simulink library "Lib_Piccolo"  (R2018b)
settings: Solver=VariableStepAuto  StartTime=0.0  StopTime=10.0  RelTol=1e-3
values from neighbouring files (symbols this model uses):
  AccelErrInt2Brakes = 0.15    [SimulationControlConfig16P.m]    (also in SimulationControlConfig16P_LEGACY.m; SimulationControlConfigTAILLESS.m = 0.2; SimulationControlConfigUTAIL.m = 0.2)
  AileronMax = 25    [SimulationControlConfig16P.m]    (also in SimulationControlConfig16P_LEGACY.m; SimulationControlConfigTAILLESS.m; SimulationControlConfigUTAIL.m)
  AileronPower = 0.00268    [SimulationControlConfig16P.m]    (also in SimulationControlConfig16P_LEGACY.m; SimulationControlConfigTAILLESS.m; SimulationControlConfigUTAIL.m)
  AileronSurfaceMax = 45    [SimulationControlConfig16P.m]    (also in SimulationControlConfig16P_LEGACY.m)
  AileronTrim = 0    [SimulationControlConfig16P.m]    (also in SimulationControlConfig16P_LEGACY.m; SimulationControlConfigTAILLESS.m; SimulationControlConfigUTAIL.m)
  Alt = 1000 + TerrainHeight    [SimulationStateConfig.m]
  AltCruise_m = testPlans(testIndx).terrainElevation * 0.3048 + 200    [SimulationControlConfig16P.m]    (also in SimulationControlConfigTAILLESS.m = 1083; SimulationControlConfigUTAIL.m = testPlans(testIndx).terrainElevation * 0.3048 + 152)
  AltitudeRate2PitchCmdIntegratorInit = 0.1    [SimulationControlPre.m]
  AltMax = 10000    [SimulationControlConfig16P.m]    (also in SimulationControlConfig16P_LEGACY.m; SimulationControlConfigTAILLESS.m; SimulationControlConfigUTAIL.m)
  AltMaxAccel = 1.25    [SimulationControlConfig16P.m]    (also in SimulationControlConfig16P_LEGACY.m = 0.9; SimulationControlConfigTAILLESS.m = 1.7; SimulationControlConfigUTAIL.m = 2)
  AltMin = 0    [SimulationControlConfig16P.m]    (also in SimulationControlConfig16P_LEGACY.m; SimulationControlConfigTAILLESS.m; SimulationControlConfigUTAIL.m)
  AltRateCmd2Pitch = 0.50    (= 0.5)    [SimulationControlConfig16P.m]    (also in SimulationControlConfig16P_LEGACY.m = 0.6; SimulationControlConfigTAILLESS.m = 0.2; SimulationControlConfigUTAIL.m = 0.3)
  AltRateError2Pitch = 0.40    (= 0.4)    [SimulationControlConfig16P.m]    (also in SimulationControlConfig16P_LEGACY.m; SimulationControlConfigTAILLESS.m = 0.55; SimulationControlConfigUTAIL.m = 0.55)
  AltRateErrorInt2Pitch = 0.50    (= 0.5)    [SimulationControlConfig16P.m]    (also in SimulationControlConfig16P_LEGACY.m = 0.45; SimulationControlConfigTAILLESS.m; SimulationControlConfigUTAIL.m = 0.75)
  AltRateLpfCutOff = 3    [SimulationControlConfig16P.m]    (also in SimulationControlConfig16P_LEGACY.m; SimulationControlConfigTAILLESS.m = 2; SimulationControlConfigUTAIL.m = 2)
  AutoNosegear2Rudder = 26    [SimulationControlConfig16P.m]    (also in SimulationControlConfig16P_LEGACY.m; SimulationControlConfigTAILLESS.m = 25.2; SimulationControlConfigUTAIL.m = 14)
  b = 5.54    [SimulationControlConfig16P.m]    (also in SimulationControlConfig16P_LEGACY.m; SimulationControlConfigTAILLESS.m = 2.37; SimulationControlConfigUTAIL.m = 2.37)
  Bank2AileronIntegratorInit = 0    [SimulationControlPre.m]
  BankMax_User = BankMax_User/180*pi    (= 0.523598775598)    [SimulationControlConfig16P.m]    (also in SimulationControlConfig16P_LEGACY.m; SimulationControlConfigTAILLESS.m = 0.610865238198; SimulationControlConfigUTAIL.m = 0.628318530718)
  baseLegFlaps = 20    [SimulationControlConfig16P.m]    (also in SimulationControlConfig16P_LEGACY.m = 0; SimulationControlConfigTAILLESS.m = 15; SimulationControlConfigUTAIL.m = 10)
  C = GeneticOpt.C    [SimulationCostFunction.m]
  c = Sw/b    (= 0.841696750903)    [SimulationControlConfig16P.m]    (also in SimulationControlConfig16P_LEGACY.m; SimulationControlConfigTAILLESS.m = 0.354008438819; SimulationControlConfigUTAIL.m = 0.354008438819)
  cell2WheelFactorMG = 5.98    [SimulationSensorConfig16P_LEGACY.m]
  cell2WheelFactorNG = 1    [SimulationSensorConfig16P_LEGACY.m]
  cellSatMaxMG = 15000    [SimulationSensorConfig16P.m]    (also in SimulationSensorConfig16P_LEGACY.m; SimulationSensorConfigTAILLESS7P.m; SimulationSensorConfigUTAIL7P.m)
  cellSatMaxNG = 1000    [SimulationSensorConfig16P.m]    (also in SimulationSensorConfig16P_LEGACY.m; SimulationSensorConfigTAILLESS7P.m; SimulationSensorConfigUTAIL7P.m)
  cellSatMinMG = -15000    [SimulationSensorConfig16P.m]    (also in SimulationSensorConfig16P_LEGACY.m; SimulationSensorConfigTAILLESS7P.m; SimulationSensorConfigUTAIL7P.m)
  cellSatMinNG = -1000    [SimulationSensorConfig16P.m]    (also in SimulationSensorConfig16P_LEGACY.m; SimulationSensorConfigTAILLESS7P.m; SimulationSensorConfigUTAIL7P.m)
  CL_Limit = CL_Max    (= 0.54)    [SimulationControlConfig16P.m]    (also in SimulationControlConfig16P_LEGACY.m; SimulationControlConfigTAILLESS.m; SimulationControlConfigUTAIL.m = 0.53)
  CL_Max = 0.54    [SimulationControlConfig16P.m]    (also in SimulationControlConfig16P_LEGACY.m; SimulationControlConfigTAILLESS.m; SimulationControlConfigUTAIL.m = 0.53)
  CL_Max_Nom = 0.465    [SimulationControlConfig16P.m]    (also in SimulationControlConfig16P_LEGACY.m; SimulationControlConfigTAILLESS.m = 0.39; SimulationControlConfigUTAIL.m)
  CL_Min = 0    [SimulationControlConfig16P.m]    (also in SimulationControlConfig16P_LEGACY.m; SimulationControlConfigTAILLESS.m; SimulationControlConfigUTAIL.m)
  ClimbMaxFraction = 0.35    [SimulationControlConfig16P.m]    (also in SimulationControlConfig16P_LEGACY.m = 0.24; SimulationControlConfigTAILLESS.m = 0.19; SimulationControlConfigUTAIL.m = 0.21)
  ClimboutMaxBank = 7.0    (= 7)    [SimulationControlConfig16P.m]    (also in SimulationControlConfig16P_LEGACY.m; SimulationControlConfigTAILLESS.m = 5; SimulationControlConfigUTAIL.m)
  ClimboutTimer = 7.0    (= 7)    [SimulationControlConfig16P.m]    (also in SimulationControlConfig16P_LEGACY.m; SimulationControlConfigTAILLESS.m; SimulationControlConfigUTAIL.m)
  dCl_per_dFlap = 0.005581818    [SimulationControlConfig16P.m]    (also in SimulationControlConfig16P_LEGACY.m = 0; SimulationControlConfigTAILLESS.m = 0; SimulationControlConfigUTAIL.m = 0)
  DecelerationCmd = 3.1    [SimulationControlConfig16P.m]    (also in SimulationControlConfig16P_LEGACY.m; SimulationControlConfigTAILLESS.m = 0.1; SimulationControlConfigUTAIL.m = 0.1)
  DeRotateLogicEndTimer = abs((NoseDownLimit_Deg-1)/DeRotateRamp_Dps)    [SimulationControlConfig16P.m]    (also in SimulationControlConfig16P_LEGACY.m; SimulationControlConfigTAILLESS.m; SimulationControlConfigUTAIL.m)
  DeRotateLogicHoldNoseUpTimer = 0.1    [SimulationControlConfig16P.m]    (also in SimulationControlConfig16P_LEGACY.m; SimulationControlConfigTAILLESS.m; SimulationControlConfigUTAIL.m)
  DeRotateLogicTimerTimeout = 2    [SimulationControlConfig16P.m]    (also in SimulationControlConfig16P_LEGACY.m; SimulationControlConfigTAILLESS.m; SimulationControlConfigUTAIL.m)
  DeRotateLowerCmdSaturation = 0    [SimulationControlConfig16P.m]    (also in SimulationControlConfig16P_LEGACY.m; SimulationControlConfigTAILLESS.m; SimulationControlConfigUTAIL.m)
  DeRotateRamp_Dps = 3    [SimulationControlConfig16P.m]    (also in SimulationControlConfig16P_LEGACY.m; SimulationControlConfigTAILLESS.m = 8; SimulationControlConfigUTAIL.m = 8)
  DeRotateUpperCmdSaturation = 7    [SimulationControlConfig16P.m]    (also in SimulationControlConfig16P_LEGACY.m; SimulationControlConfigTAILLESS.m; SimulationControlConfigUTAIL.m)
  DescentMaxFraction = 0.22    [SimulationControlConfig16P.m]    (also in SimulationControlConfig16P_LEGACY.m = 0.2; SimulationControlConfigTAILLESS.m = 0.17; SimulationControlConfigUTAIL.m = 0.17)
  DesktopSimTerrainOffset_m = 0.406    [SimulationAircraftConfig.m]
  downwindFlaps = 0    [SimulationControlConfig16P.m]    (also in SimulationControlConfig16P_LEGACY.m; SimulationControlConfigTAILLESS.m; SimulationControlConfigUTAIL.m)
  DP_init = 0.5*1.225*V_init^2    [SimulationControlConfig16P.m]    (also in SimulationControlConfig16P_LEGACY.m; SimulationControlConfigTAILLESS.m; SimulationControlConfigUTAIL.m)
  dscNoiseMG = 1    [SimulationSensorConfig16P_LEGACY.m]
  dscNoiseNG = 0.25    [SimulationSensorConfig16P_LEGACY.m]
  DSCnumBits = 24    [SimulationSensorConfig16P.m]    (also in SimulationSensorConfig16P_LEGACY.m; SimulationSensorConfigTAILLESS7P.m; SimulationSensorConfigUTAIL7P.m)
  DSCRangeMaxMG = 15000    [SimulationSensorConfig16P.m]    (also in SimulationSensorConfig16P_LEGACY.m; SimulationSensorConfigTAILLESS7P.m; SimulationSensorConfigUTAIL7P.m)
  DSCRangeMaxNG = 1000    [SimulationSensorConfig16P.m]    (also in SimulationSensorConfig16P_LEGACY.m; SimulationSensorConfigTAILLESS7P.m; SimulationSensorConfigUTAIL7P.m)
  DSCRangeMinMG = -15000    [SimulationSensorConfig16P.m]    (also in SimulationSensorConfig16P_LEGACY.m; SimulationSensorConfigTAILLESS7P.m; SimulationSensorConfigUTAIL7P.m)
  DSCRangeMinNG = -1000    [SimulationSensorConfig16P.m]    (also in SimulationSensorConfig16P_LEGACY.m; SimulationSensorConfigTAILLESS7P.m; SimulationSensorConfigUTAIL7P.m)
  dt = DLLSim.dt    [SimulationTimeStep.m]    (also in SimulationTrim.m = 0.02)
  EarlyTouchdownThreshold = 3.0    (= 3)    [SimulationControlConfig16P.m]    (also in SimulationControlConfig16P_LEGACY.m; SimulationControlConfigTAILLESS.m = 2.2; SimulationControlConfigUTAIL.m = 2.5)
  ElevatorDeflectionRate = 15    [SimulationControlConfig16P.m]    (also in SimulationControlConfig16P_LEGACY.m = 12; SimulationControlConfigTAILLESS.m = 10; SimulationControlConfigUTAIL.m = 12)
  ElevatorMax = 25    [SimulationControlConfig16P.m]    (also in SimulationControlConfig16P_LEGACY.m; SimulationControlConfigTAILLESS.m; SimulationControlConfigUTAIL.m)
  ElevatorPower = -0.002209    [SimulationControlConfig16P.m]    (also in SimulationControlConfig16P_LEGACY.m; SimulationControlConfigTAILLESS.m = -0.002956; SimulationControlConfigUTAIL.m = -0.00205983)
  ElevatorTrim = -3.5    [SimulationControlConfig16P.m]    (also in SimulationControlConfig16P_LEGACY.m; SimulationControlConfigTAILLESS.m = -6; SimulationControlConfigUTAIL.m = -8)
  elevonBias = 0    [SimulationControlConfig16P.m]    (also in SimulationControlConfig16P_LEGACY.m; SimulationControlConfigTAILLESS.m; SimulationControlConfigUTAIL.m)
  Enable_TAS_Protection = 0    [SimulationControlConfig16P.m]    (also in SimulationControlConfig16P_LEGACY.m; SimulationControlConfigTAILLESS.m; SimulationControlConfigUTAIL.m)
  EnableCrossTrackAbort = 1    [SimulationControlConfig16P.m]    (also in SimulationControlConfigTAILLESS.m; SimulationControlConfigUTAIL.m)
  EnergyBandwidth = 0.02    [SimulationControlConfig16P.m]    (also in SimulationControlConfig16P_LEGACY.m; SimulationControlConfigTAILLESS.m = 0.06; SimulationControlConfigUTAIL.m = 0.06)
  EngineLhFuelCut = 0    [SimulationAircraftConfig.m]
  EngineRhFuelCut = 0    [SimulationAircraftConfig.m]
  FastThrottleRate = 0.075    [SimulationControlConfig16P.m]    (also in SimulationControlConfig16P_LEGACY.m = 0.05; SimulationControlConfigTAILLESS.m = 0.1; SimulationControlConfigUTAIL.m = 0.1)
  FilterWarmUpTime = 2    [SimulationSensorConfig16P.m]    (also in SimulationSensorConfig16P_LEGACY.m; SimulationSensorConfigTAILLESS7P.m; SimulationSensorConfigUTAIL7P.m)
  finalApproachFlaps = 20    [SimulationControlConfig16P.m]    (also in SimulationControlConfig16P_LEGACY.m = 0; SimulationControlConfigTAILLESS.m = 22; SimulationControlConfigUTAIL.m = 10)
  FinalDescentSlope_Deg = testPlans(testIndx).descentSlope    [SimulationControlConfig16P.m]    (also in SimulationControlConfig16P_LEGACY.m; SimulationControlConfigTAILLESS.m; SimulationControlConfigUTAIL.m)
  flapMax = 0    [SimulationControlConfig16P.m]    (also in SimulationControlConfig16P_LEGACY.m; SimulationControlConfigTAILLESS.m; SimulationControlConfigUTAIL.m)
  flapRate = 7.5    [SimulationControlConfig16P.m]    (also in SimulationControlConfig16P_LEGACY.m; SimulationControlConfigTAILLESS.m = 6.6; SimulationControlConfigUTAIL.m)
  FlareHeight = 5    [SimulationControlConfig16P.m]    (also in SimulationControlConfig16P_LEGACY.m = 4.8; SimulationControlConfigTAILLESS.m = 2.5; SimulationControlConfigUTAIL.m = 2)
  FlareVerticalRate_mps = -0.4    [SimulationControlConfig16P.m]    (also in SimulationControlConfig16P_LEGACY.m = -0.5; SimulationControlConfigTAILLESS.m = -0.15; SimulationControlConfigUTAIL.m = -0.15)
  Fp_Aileron = 0.55*2*pi*RollRateLpfCutoff*dt    [SimulationControlConfig16P.m]    (also in SimulationControlConfig16P_LEGACY.m; SimulationControlConfigTAILLESS.m; SimulationControlConfigUTAIL.m)
  Fp_Alt = 0.55*AltBandwidth    (= 0.099)    [SimulationControlConfig16P.m]    (also in SimulationControlConfig16P_LEGACY.m; SimulationControlConfigTAILLESS.m = 0.587477826221; SimulationControlConfigUTAIL.m = 0.69115038379)
  Fp_AltRate = 0.55*2*pi*AltRateLpfCutOff*dt    [SimulationControlConfig16P.m]    (also in SimulationControlConfig16P_LEGACY.m; SimulationControlConfigTAILLESS.m; SimulationControlConfigUTAIL.m)
  Fp_Elevator = 0.55*2*pi*PitchRateLpfCutoff*dt    [SimulationControlConfig16P.m]    (also in SimulationControlConfig16P_LEGACY.m; SimulationControlConfigTAILLESS.m; SimulationControlConfigUTAIL.m)
  Fp_Energy = 0.55*2*pi*EnergyBandwidth    (= 0.069115038379)    [SimulationControlConfig16P.m]    (also in SimulationControlConfig16P_LEGACY.m; SimulationControlConfigTAILLESS.m = 0.207345115137; SimulationControlConfigUTAIL.m = 0.207345115137)
  Fp_Energy2 = 0.55*2*pi*EnergyBandwidth*dt    [SimulationControlConfig16P.m]    (also in SimulationControlConfig16P_LEGACY.m; SimulationControlConfigTAILLESS.m; SimulationControlConfigUTAIL.m)
  Fp_Pitch = 0.55*2*pi*PitchBandwidth    (= 2.76460153516)    [SimulationControlConfig16P.m]    (also in SimulationControlConfig16P_LEGACY.m = 3.11017672705; SimulationControlConfigTAILLESS.m = 3.80132711084; SimulationControlConfigUTAIL.m = 2.41902634326)
  Fp_Pitch_2 = 0.55*2*pi*PitchBandwidth*dt    [SimulationControlConfig16P.m]    (also in SimulationControlConfig16P_LEGACY.m; SimulationControlConfigTAILLESS.m; SimulationControlConfigUTAIL.m)
  Fp_Roll = RollBandwidth^2    (= 1)    [SimulationControlConfig16P.m]    (also in SimulationControlConfig16P_LEGACY.m = 1.44; SimulationControlConfigTAILLESS.m; SimulationControlConfigUTAIL.m)
  Fp_Rudder = 0.55*2*pi*YawRateLpfCutoff*dt    [SimulationControlConfig16P.m]    (also in SimulationControlConfig16P_LEGACY.m; SimulationControlConfigTAILLESS.m; SimulationControlConfigUTAIL.m)
  Fp_TAS = 0.55*2*pi*TASBandwidth    (= 0.103672557568)    [SimulationControlConfig16P.m]    (also in SimulationControlConfig16P_LEGACY.m; SimulationControlConfigTAILLESS.m = 0.172787595947; SimulationControlConfigUTAIL.m = 0.172787595947)
  Fp_TAS_Filter = 2*pi*TasLpfCutoff*dt    [SimulationControlConfig16P.m]    (also in SimulationControlConfig16P_LEGACY.m; SimulationControlConfigTAILLESS.m; SimulationControlConfigUTAIL.m)
  Fp_Turn = 0.55*2*pi*TurnErrLPFcutoff    (= 0.0345575191895)    [SimulationControlConfig16P.m]    (also in SimulationControlConfig16P_LEGACY.m; SimulationControlConfigTAILLESS.m = 0.172787595947; SimulationControlConfigUTAIL.m = 0.172787595947)
  Fp_TurnDerr = 0.55*2*pi*TurnDerivativeLPFcutoff    (= 0.0345575191895)    [SimulationControlConfig16P.m]    (also in SimulationControlConfig16P_LEGACY.m; SimulationControlConfigTAILLESS.m = 0.172787595947; SimulationControlConfigUTAIL.m = 0.172787595947)
  FTV = 3    [SimulationAircraftConfig.m]
  ftvStaticPositionError = 1/1.18    (= 0.847457627119)    [SimulationSensorConfig16P.m]    (also in SimulationSensorConfig16P_LEGACY.m; SimulationSensorConfigTAILLESS7P.m = 1; SimulationSensorConfigUTAIL7P.m = 1)
  g = 9.81    [SimulationStateConfig.m]
  GustSpd_Kts = testPlans(testIndx).gustSpd    [SimulationStateConfig.m]
  GustTriggerVal = testPlans(testIndx).gustTriggerVal    [SimulationStateConfig.m]
  HeadingErr2TurnRate = 0.5    [SimulationControlConfig16P.m]    (also in SimulationControlConfig16P_LEGACY.m; SimulationControlConfigTAILLESS.m; SimulationControlConfigUTAIL.m)
  HeadingErrDer2TurnRate = 0.3    [SimulationControlConfig16P.m]    (also in SimulationControlConfig16P_LEGACY.m; SimulationControlConfigTAILLESS.m; SimulationControlConfigUTAIL.m)
  IASbounce = IASstall*0.8    [SimulationControlPre.m]
  IAScruiseCMD = sqrt(2*m*9.81/(1.225*Sw*CL_cruise))    [SimulationControlConfig16P.m]    (also in SimulationControlConfig16P_LEGACY.m; SimulationControlConfigTAILLESS.m; SimulationControlConfigUTAIL.m)
  IASfinalCMD = 1.12 * IASmin    [SimulationControlConfig16P.m]    (also in SimulationControlConfig16P_LEGACY.m = 1.10 * IASmin; SimulationControlConfigTAILLESS.m = 1.10 * IASmin; SimulationControlConfigUTAIL.m = 1.15 * IASmin)
  IASflareCMD = IASstall    [SimulationControlConfig16P.m]    (also in SimulationControlConfig16P_LEGACY.m; SimulationControlConfigTAILLESS.m; SimulationControlConfigUTAIL.m)
  IASmax = 64    [SimulationControlConfig16P.m]    (also in SimulationControlConfig16P_LEGACY.m = 46; SimulationControlConfigTAILLESS.m = 38.58; SimulationControlConfigUTAIL.m = 35)
  IASmin = sqrt(2*m*9.81/(1.225*Sw*0.9*CL_Max_Nom))    [SimulationControlConfig16P.m]    (also in SimulationControlConfig16P_LEGACY.m; SimulationControlConfigTAILLESS.m; SimulationControlConfigUTAIL.m)
  IASshortCMD = IASstall    [SimulationControlConfig16P.m]    (also in SimulationControlConfig16P_LEGACY.m; SimulationControlConfigTAILLESS.m; SimulationControlConfigUTAIL.m)
  IASstall = sqrt(2*m*9.81/(1.225*Sw*CL_Max))    [SimulationControlConfig16P.m]    (also in SimulationControlConfig16P_LEGACY.m; SimulationControlConfigTAILLESS.m; SimulationControlConfigUTAIL.m)
  inFlight = 1    [SimulationControlConfig16P.m]    (also in SimulationControlConfigTAILLESS.m; SimulationControlConfigUTAIL.m)
  JetCatOffset = 5    [SimulationControlConfig16P.m]    (also in SimulationControlConfig16P_LEGACY.m)
  LaunchRollingElevator = -1.5    [SimulationControlConfig16P.m]    (also in SimulationControlConfig16P_LEGACY.m; SimulationControlConfigTAILLESS.m = 1; SimulationControlConfigUTAIL.m = 1)
  ldg_NosegearMax = 10    [SimulationControlConfig16P.m]    (also in SimulationControlConfig16P_LEGACY.m; SimulationControlConfigTAILLESS.m; SimulationControlConfigUTAIL.m)
  ldg_TrackVyErrInt2Nosegear = 0.1250    (= 0.125)    [SimulationControlConfig16P.m]    (also in SimulationControlConfig16P_LEGACY.m; SimulationControlConfigTAILLESS.m = 0.00714285714286; SimulationControlConfigUTAIL.m = 0.00714285714286)
  ldg_TrackVyErrPro2Nosegear = 0.35    [SimulationControlConfig16P.m]    (also in SimulationControlConfig16P_LEGACY.m; SimulationControlConfigTAILLESS.m = 0.0546666666667; SimulationControlConfigUTAIL.m = 0.0546666666667)
  ldg_TrackY2Vy = 0.07    [SimulationControlConfig16P.m]    (also in SimulationControlConfig16P_LEGACY.m; SimulationControlConfigTAILLESS.m = 0.17; SimulationControlConfigUTAIL.m = 0.17)
  ldg_Vy2NosegearScalingPower = 1.075    [SimulationControlConfig16P.m]    (also in SimulationControlConfig16P_LEGACY.m; SimulationControlConfigTAILLESS.m = 0.6; SimulationControlConfigUTAIL.m = 0.5)
  ldg_Y2VyScalingPower = 0.175    [SimulationControlConfig16P.m]    (also in SimulationControlConfig16P_LEGACY.m; SimulationControlConfigTAILLESS.m = 0; SimulationControlConfigUTAIL.m = 0)
  ldg_YawRate2Nosegear = 0.175    [SimulationControlConfig16P.m]    (also in SimulationControlConfig16P_LEGACY.m; SimulationControlConfigTAILLESS.m = 0.065; SimulationControlConfigUTAIL.m = 0.065)
  LiftSlope = 0.064285    [SimulationControlConfig16P.m]    (also in SimulationControlConfig16P_LEGACY.m; SimulationControlConfigTAILLESS.m = 0.058631; SimulationControlConfigUTAIL.m)
  LPFaileronInit = 0    [SimulationControlPre.m]
  LPFclestInit = 0    [SimulationControlPre.m]
  LPFenergyFFInit = 0    [SimulationControlPre.m]
  LPFtasInit = V_init + 2    [SimulationControlPre.m]
  LPFthrottleInit = ThrottleTrim    [SimulationControlPre.m]
  LPFturnErrInit = 0    [SimulationControlPre.m]
  ... (+115 more)
undefined symbols (not defined in the file or in its folder): abortFlag, alphaHPF, apmDelay, BRWNOUT, CRAWOR, CRAWUR, DiscIntNeverNeededParam, DLLSim, DLLSimStep, ECOMOR, ECOMUR, Fp_Tas, GustTrigger_HeightAgl_m, IPSTAT, LCINTEG, Ldg_Persist_Time, LOWER_FLAGS, MSG_ENABLE, NoiseStd, OLDVAL, OVERRIDE_ENABLE, OVERRIDE_VALUE, REBOOT, reversionEnable, revIASMax, revIASMin, revPitchMax, revPitchMin, revPitchRateMax, revRollMax, revRollRateMax, SAMPLE, SCALON, SensorModel, sigbuilder_block, Sim_Vx, Sim_Vy, Sim_Vz, Sim_Xpos, Sim_Ypos, Sim_Zpos, SYSOR, SYSUR, TARE, TEMPOR, TEMPUR, testIndx, testPlan, testPlans, Trim_piccoloInCmd, Trim_REFSI_FD_IN_nmodeCgShifterCmd_Ft, Trim_REFSI_FD_IN_nmodeFlapLhIBCmd_Deg, Trim_REFSI_FD_IN_nmodeFlapLhOBCmd_Deg, Trim_REFSI_FD_IN_nmodeFlapRhIBCmd_Deg, Trim_REFSI_FD_IN_nmodeFlapRhOBCmd_Deg, Trim_REFSI_FD_IN_nmodeSlatLhCmd_Deg, Trim_REFSI_FD_IN_nmodeSlatRhCmd_Deg, Trim_REFSI_FD_IN_nmodeSplrLhInbdCmd_Deg, Trim_REFSI_FD_IN_nmodeSplrLhOutbdCmd_Deg ... (+5)
libraries: simulink x866, aerolibconvert2 x60, $bdroot x52, aerolibatmos2 x5, dspswit3 x5, simulink_extras x4, dsparch4 x2, Lib_Piccolo_Alt x2, eeGeneralControl x1, dspindex x1
(part 42 of 44)

== system Lib_Piccolo/Ground Detection Systems/WoW Wrapper/Variant Subsystem/Load Cell WoW Model 20/WOW Module/Subsystem/Comms Timeout Logic ==
  MGR_STALE_LOAD : Inport  OutDataTypeStr=boolean
  MGL_STALE_LOAD : Inport  Port=2  OutDataTypeStr=boolean
  NG_STALE_LOAD : Inport  Port=3  OutDataTypeStr=boolean
  MGR_STALE_FLAG : Inport  Port=4  OutDataTypeStr=boolean
  MGL_STALE_FLAG : Inport  Port=5  OutDataTypeStr=boolean
  NG_STALE_FLAG : Inport  Port=6  OutDataTypeStr=boolean
  INIT : Inport  Port=7  OutDataTypeStr=boolean
  AND{,1..14} (15 alike) : Logic  IconShape=distinctive  AllPortsSameDT=off  OutDataTypeStr=boolean
  FLAG Timeout Counter : Subsystem
  FLAG Timeout Counter1 : $bdroot/Ground Detection Systems/WoW Wrapper/Variant Subsystem/Load Cell WoW Model 20/WOW Module/Subsystem/Comms Timeout Logic/FLAG Timeout Counter  SystemSampleTime=-1
  FLAG Timeout Counter2 : $bdroot/Ground Detection Systems/WoW Wrapper/Variant Subsystem/Load Cell WoW Model 20/WOW Module/Subsystem/Comms Timeout Logic/FLAG Timeout Counter  SystemSampleTime=-1
  LOAD Timeout Counter : Subsystem
  LOAD Timeout Counter1 : $bdroot/Ground Detection Systems/WoW Wrapper/Variant Subsystem/Load Cell WoW Model 20/WOW Module/Subsystem/Comms Timeout Logic/LOAD Timeout Counter  SystemSampleTime=-1
  LOAD Timeout Counter2 : $bdroot/Ground Detection Systems/WoW Wrapper/Variant Subsystem/Load Cell WoW Model 20/WOW Module/Subsystem/Comms Timeout Logic/LOAD Timeout Counter  SystemSampleTime=-1
  Latch : Subsystem
  Latch{1..5} (5 alike) : $bdroot/Ground Detection Systems/WoW Wrapper/Variant Subsystem/Load Cell WoW Model 20/WOW Module/Subsystem/Comms Timeout Logic/Latch  SystemSampleTime=-1
  NOT{,1..6} (7 alike) : Logic  Operator=NOT  IconShape=distinctive  AllPortsSameDT=off  OutDataTypeStr=boolean
  Reset Value Selector : Subsystem
  MGR_LOAD_TIMEOUT : Outport  OutDataTypeStr=boolean
  MGL_LOAD_TIMEOUT : Outport  Port=2  OutDataTypeStr=boolean
  NG_LOAD_TIMEOUT : Outport  Port=3  OutDataTypeStr=boolean
  MGR_FLAG_TIMEOUT : Outport  Port=4  OutDataTypeStr=boolean
  MGL_FLAG_TIMEOUT : Outport  Port=5  OutDataTypeStr=boolean
  NG_FLAG_TIMEOUT : Outport  Port=6  OutDataTypeStr=boolean
  MGR_ACTIVE : Outport  Port=7  OutDataTypeStr=boolean
  MGL_ACTIVE : Outport  Port=8  OutDataTypeStr=boolean
  NG_ACTIVE : Outport  Port=9  OutDataTypeStr=boolean
  wires:
  AND5/1 -> LOAD Timeout Counter1/1
  AND6/1 -> LOAD Timeout Counter2/1
  MGR_STALE_LOAD/1 -> NOT/1, AND4/1
  AND8/1 -> FLAG Timeout Counter1/1
  Reset Value Selector/1(Reset Value LOAD) -> LOAD Timeout Counter2/2, LOAD Timeout Counter1/2, LOAD Timeout Counter/2(x0)
  LOAD Timeout Counter2/1 -> NG_LOAD_TIMEOUT/1  "NG_LOAD_TIMEOUT"
  AND7/1 -> FLAG Timeout Counter/1(Trigger/!Rst)
  AND9/1 -> FLAG Timeout Counter2/1
  INIT/1 -> NOT1/1, Reset Value Selector/1(Init)
  AND4/1 -> LOAD Timeout Counter/1(Trigger/!Rst)
  Reset Value Selector/2(Reset Value FLAG) -> FLAG Timeout Counter2/2, FLAG Timeout Counter1/2, FLAG Timeout Counter/2(x0)
  FLAG Timeout Counter1/1 -> MGL_FLAG_TIMEOUT/1  "MGL_FLAG_TIMEOUT"
  FLAG Timeout Counter/1(TIMEOUT) -> MGR_FLAG_TIMEOUT/1  "MGR_FLAG_TIMEOUT"
  LOAD Timeout Counter1/1 -> MGL_LOAD_TIMEOUT/1  "MGL_LOAD_TIMEOUT"
  FLAG Timeout Counter2/1 -> NG_FLAG_TIMEOUT/1  "NG_FLAG_TIMEOUT"
  LOAD Timeout Counter/1(TIMEOUT) -> MGR_LOAD_TIMEOUT/1  "MGR_LOAD_TIMEOUT"
  NOT/1 -> AND1/1
  NOT2/1 -> AND2/1
  MGL_STALE_LOAD/1 -> NOT2/1, AND5/1
  NOT3/1 -> AND3/1
  NG_STALE_LOAD/1 -> NOT3/1, AND6/1
  NOT4/1 -> AND10/1
  MGR_STALE_FLAG/1 -> NOT4/1, AND7/1
  NOT5/1 -> AND11/1
  MGL_STALE_FLAG/1 -> NOT5/1, AND8/1
  NOT6/1 -> AND12/1
  NG_STALE_FLAG/1 -> NOT6/1, AND9/1
  NOT1/1 -> AND1/2, Latch/2(Enable/!Rst), AND4/2, AND2/2, Latch1/2, AND5/2, AND3/2, Latch2/2, AND6/2, AND10/2, Latch3/2, AND7/2, AND11/2, Latch4/2, AND8/2, AND12/2, Latch5/2, AND9/2
  AND1/1 -> Latch/1(D)
  AND2/1 -> Latch1/1
  AND3/1 -> Latch2/1
  AND10/1 -> Latch3/1
  Latch/1(Q_Latched) -> AND/1  "MGR_LOAD_ACTIVE"
  AND11/1 -> Latch4/1
  AND12/1 -> Latch5/1
  Latch1/1 -> AND13/1  "MGL_LOAD_ACTIVE"
  Latch2/1 -> AND14/1  "NG_LOAD_ACTIVE"
  Latch3/1 -> AND/2  "MGR_FLAG_ACTIVE"
  Latch4/1 -> AND13/2  "MGL_FLAG_ACTIVE"
  Latch5/1 -> AND14/2  "NG_FLAG_ACTIVE"
  AND/1 -> MGR_ACTIVE/1
  AND13/1 -> MGL_ACTIVE/1
  AND14/1 -> NG_ACTIVE/1

== system Lib_Piccolo/Ground Detection Systems/WoW Wrapper/Variant Subsystem/Load Cell WoW Model 20/WOW Module/Subsystem/Health Check ==
  PIC_AP_MODE : Inport  OutDataTypeStr=uint8
  MGR FLAG Word : Inport  Port=2  OutDataTypeStr=uint16
  MGR STAT Word : Inport  Port=3  OutDataTypeStr=uint16
  MGL FLAG Word : Inport  Port=4  OutDataTypeStr=uint16
  MGL STAT Word : Inport  Port=5  OutDataTypeStr=uint16
  NG FLAG Word : Inport  Port=6  OutDataTypeStr=uint16
  NG STAT Word : Inport  Port=7  OutDataTypeStr=uint16
  MGR_LOAD_TIMEOUT : Inport  Port=8  OutDataTypeStr=boolean
  MGL_LOAD_TIMEOUT : Inport  Port=9  OutDataTypeStr=boolean
  NG_LOAD_TIMEOUT : Inport  Port=10  OutDataTypeStr=boolean
  MGR_FLAG_TIMEOUT : Inport  Port=11  OutDataTypeStr=boolean
  MGL_FLAG_TIMEOUT : Inport  Port=12  OutDataTypeStr=boolean
  NG_FLAG_TIMEOUT : Inport  Port=13  OutDataTypeStr=boolean
  WOW_N : Inport  Port=14
  Bus Selector : BusSelector  OutputSignals=WOW_MGR_N,WOW_MGL_N,WOW_NG_N
  DSC FLAG Decode : Subsystem
  DSC STAT Decode : Subsystem
  MGL DSC Fail Logic : $bdroot/Ground Detection Systems/WoW Wrapper/Variant Subsystem/Load Cell WoW Model 20/WOW Module/Subsystem/Health Check/MGR DSC Fail Logic  SystemSampleTime=-1
  MGR DSC Fail Logic : Subsystem
  NG DSC Fail Logic : Subsystem
  MGR_FAIL : Outport  OutDataTypeStr=boolean
  MGL_FAIL : Outport  Port=2  OutDataTypeStr=boolean
  NG_FAIL : Outport  Port=3  OutDataTypeStr=boolean
  MGR_FLAGS : Outport  Port=4  OutDataTypeStr=Bus: FLAG_SIGNAL_BUS
  MGL_FLAGS : Outport  Port=5  OutDataTypeStr=Bus: FLAG_SIGNAL_BUS
  NG_FLAGS : Outport  Port=6  OutDataTypeStr=Bus: FLAG_SIGNAL_BUS
  MGR_HEALTH : Outport  Port=7  OutDataTypeStr=Bus: HEALTH_SIGNAL_BUS
  MGL_HEALTH : Outport  Port=8  OutDataTypeStr=Bus: HEALTH_SIGNAL_BUS
  NG_HEALTH : Outport  Port=9  OutDataTypeStr=Bus: HEALTH_SIGNAL_BUS
  MGR_STAT : Outport  Port=10  OutDataTypeStr=Bus: STAT_SIGNAL_BUS
  MGL_STAT : Outport  Port=11  OutDataTypeStr=Bus: STAT_SIGNAL_BUS
  NG_STAT : Outport  Port=12  OutDataTypeStr=Bus: STAT_SIGNAL_BUS
  wires:
  DSC FLAG Decode/1(MGR_FLAG_RESET) -> MGR DSC Fail Logic/4(FLAG_RESET)  "MGR_FLAG_RESET"
  NG FLAG Word/1 -> DSC FLAG Decode/3(NG FLAG Word)
  DSC FLAG Decode/6(NG_FLAGS) -> NG_FLAGS/1  "NG_FLAGS"
  DSC FLAG Decode/4(MGR_FLAGS) -> MGR_FLAGS/1  "MGR_FLAGS"
  DSC FLAG Decode/5(MGL_FLAGS) -> MGL_FLAGS/1  "MGL_FLAGS"
  MGL FLAG Word/1 -> DSC FLAG Decode/2(MGL FLAG Word)
  DSC FLAG Decode/2(MGL_FLAG_RESET) -> MGL DSC Fail Logic/4  "MGL_FLAG_RESET"
  DSC FLAG Decode/3(NG_FLAG_RESET) -> NG DSC Fail Logic/4(FLAG_RESET)  "NG_FLAG_RESET"
  MGR FLAG Word/1 -> DSC FLAG Decode/1(MGR FLAG Word)
  MGR_LOAD_TIMEOUT/1 -> MGR DSC Fail Logic/3(LOAD_TIMEOUT)
  MGL_LOAD_TIMEOUT/1 -> MGL DSC Fail Logic/3
  NG_LOAD_TIMEOUT/1 -> NG DSC Fail Logic/3(LOAD_TIMEOUT)
  MGR DSC Fail Logic/1(DSC_FAIL) -> MGR_FAIL/1  "MGR_DSC_FAIL"
  MGL DSC Fail Logic/1 -> MGL_FAIL/1  "MGL_DSC_FAIL"
  NG DSC Fail Logic/1(DSC_FAIL) -> NG_FAIL/1  "NG_DSC_FAIL"
  MGR DSC Fail Logic/2(MGR_HEALTH) -> MGR_HEALTH/1  "MGR_HEALTH"
  MGL DSC Fail Logic/2 -> MGL_HEALTH/1  "MGL_HEALTH"
  NG DSC Fail Logic/2(MGR_HEALTH) -> NG_HEALTH/1  "NG_HEALTH"
  WOW_N/1 -> Bus Selector/1
  Bus Selector/1 -> MGR DSC Fail Logic/2(WOW_N)  "<WOW_MGR_N>"
  Bus Selector/2 -> MGL DSC Fail Logic/2  "<WOW_MGL_N>"
  Bus Selector/3 -> NG DSC Fail Logic/2(WOW_N)  "<WOW_NG_N>"
  MGL STAT Word/1 -> DSC STAT Decode/2(MGL STAT Word)
  NG STAT Word/1 -> DSC STAT Decode/3(NG STAT Word)
  MGR STAT Word/1 -> DSC STAT Decode/1(MGR STAT Word)
  DSC STAT Decode/1(MGR_STAT) -> MGR_STAT/1
  DSC STAT Decode/2(MGL_STAT) -> MGL_STAT/1
  DSC STAT Decode/3(NG_STAT) -> NG_STAT/1
  PIC_AP_MODE/1 -> NG DSC Fail Logic/1(PIC_AP_MODE), MGL DSC Fail Logic/1, MGR DSC Fail Logic/1(PIC_AP_MODE)
  MGR_FLAG_TIMEOUT/1 -> MGR DSC Fail Logic/5(FLAG_TIMEOUT)
  MGL_FLAG_TIMEOUT/1 -> MGL DSC Fail Logic/5
  NG_FLAG_TIMEOUT/1 -> NG DSC Fail Logic/5(FLAG_TIMEOUT)

== system Lib_Piccolo/Ground Detection Systems/WoW Wrapper/Variant Subsystem/Load Cell WoW Model 20/WOW Module/T//O Configuration/Latch ==
  D : Inport
  Enable/!Rst : Inport  Port=2
  AND : Logic  IconShape=distinctive  AllPortsSameDT=off  OutDataTypeStr=boolean
  Constant : Constant  OutDataTypeStr=boolean
  OR : Logic  Operator=OR  IconShape=distinctive  AllPortsSameDT=off  OutDataTypeStr=boolean
  Switch : Switch  Criteria=u2 > Threshold  Threshold=0.5
  Unit Delay : UnitDelay  SampleTime=-1
  Q_Latched : Outport
  wires:
  Unit Delay/1 -> OR/2
  Switch/1 -> Q_Latched/1, Unit Delay/1
  D/1 -> Switch/3, OR/1
  OR/1 -> AND/1
  AND/1 -> Switch/2
  Enable/!Rst/1 -> AND/2
  Constant/1 -> Switch/1

== system Lib_Piccolo/Ground Detection Systems/WoW Wrapper/Variant Subsystem/Load Cell WoW Model 20/WOW Module/T//O Configuration/Latch Timer ==
  Enable/!Rst : Inport
  Compare To Constant1 : simulink/Logic and Bit Operations/Compare To Constant  relop=>  const=0  OutDataTypeStr=uint8
  Compare To Constant2 : simulink/Logic and Bit Operations/Compare To Constant  relop=>=  const=period  OutDataTypeStr=boolean
  Compare To Constant3 : simulink/Logic and Bit Operations/Compare To Constant  relop===  const=0  OutDataTypeStr=boolean
  Discrete-Time Integrator : DiscreteIntegrator  ExternalReset=level  SampleTime=-1  OutDataTypeStr=double  ICPrevOutput=DiscIntNeverNeededParam  ICPrevScaledInput=DiscIntNeverNeededParam
  Expired : Outport
  wires:
  Compare To Constant3/1 -> Discrete-Time Integrator/2
  Enable/!Rst/1 -> Compare To Constant3/1, Compare To Constant1/1
  Discrete-Time Integrator/1 -> Compare To Constant2/1
  Compare To Constant2/1 -> Expired/1
  Compare To Constant1/1 -> Discrete-Time Integrator/1

== system Lib_Piccolo/Ground Detection Systems/WoW Wrapper/Variant Subsystem/Load Cell WoW Model 20/WOW Module/T//O Configuration/Persistance Timer ==
  Enable/!Rst : Inport
  Compare To Constant1 : simulink/Logic and Bit Operations/Compare To Constant  relop=>  const=0  OutDataTypeStr=uint8
  Compare To Constant2 : simulink/Logic and Bit Operations/Compare To Constant  relop=>=  const=period  OutDataTypeStr=boolean
  Compare To Constant3 : simulink/Logic and Bit Operations/Compare To Constant  relop===  const=0  OutDataTypeStr=boolean
  Discrete-Time Integrator : DiscreteIntegrator  ExternalReset=level  SampleTime=-1  OutDataTypeStr=double  ICPrevOutput=DiscIntNeverNeededParam  ICPrevScaledInput=DiscIntNeverNeededParam
  Expired : Outport
  wires:
  Compare To Constant3/1 -> Discrete-Time Integrator/2
  Enable/!Rst/1 -> Compare To Constant3/1, Compare To Constant1/1
  Discrete-Time Integrator/1 -> Compare To Constant2/1
  Compare To Constant2/1 -> Expired/1
  Compare To Constant1/1 -> Discrete-Time Integrator/1

== system Lib_Piccolo/Ground Detection Systems/WoW Wrapper/Variant Subsystem/Load Cell WoW Model 1/Landing Configuration/Latch Timer Selection/Latch Timer Selection/Timer Select Latch ==
  D : Inport
  Enable/!Rst : Inport  Port=2
  AND : Logic  IconShape=distinctive  AllPortsSameDT=off  OutDataTypeStr=boolean
  Constant : Constant
  OR : Logic  Operator=OR  IconShape=distinctive  AllPortsSameDT=off  OutDataTypeStr=boolean
  Switch : Switch  Criteria=u2 > Threshold  Threshold=0.5
  Unit Delay : UnitDelay  SampleTime=-1
  Q_Latched : Outport
  wires:
  Unit Delay/1 -> OR/2
  Switch/1 -> Q_Latched/1, Unit Delay/1
  D/1 -> Switch/3, OR/1
  OR/1 -> AND/1
  AND/1 -> Switch/2
  Enable/!Rst/1 -> AND/2
  Constant/1 -> Switch/1

== system Lib_Piccolo/Ground Detection Systems/WoW Wrapper/Variant Subsystem/Load Cell WoW Model 1 16P5 AsFlown 2022/Landing Configuration/Latch Timer Selection/Latch Timer Selection/Timer Select Latch ==
  D : Inport
  Enable/!Rst : Inport  Port=2
  AND : Logic  IconShape=distinctive  AllPortsSameDT=off  OutDataTypeStr=boolean
  Constant : Constant
  OR : Logic  Operator=OR  IconShape=distinctive  AllPortsSameDT=off  OutDataTypeStr=boolean
  Switch : Switch  Criteria=u2 > Threshold  Threshold=0.5
  Unit Delay : UnitDelay  SampleTime=-1
  Q_Latched : Outport
  wires:
  Constant/1 -> Switch/1
  Enable/!Rst/1 -> AND/2
  AND/1 -> Switch/2
  OR/1 -> AND/1
  D/1 -> OR/1, Switch/3
  Switch/1 -> Unit Delay/1, Q_Latched/1
  Unit Delay/1 -> OR/2

== system Lib_Piccolo/Ground Detection Systems/WoW Wrapper/Variant Subsystem/Load Cell WoW Model 1 7P AsFlown/Landing Configuration/Latch Timer Selection/Latch Timer Selection/Timer Select Latch ==
  D : Inport
  Enable/!Rst : Inport  Port=2
  AND : Logic  IconShape=distinctive  AllPortsSameDT=off  OutDataTypeStr=boolean
  Constant : Constant
  OR : Logic  Operator=OR  IconShape=distinctive  AllPortsSameDT=off  OutDataTypeStr=boolean
  Switch : Switch  Criteria=u2 > Threshold  Threshold=0.5
  Unit Delay : UnitDelay  SampleTime=-1
  Q_Latched : Outport
  wires:
  Unit Delay/1 -> OR/2
  Switch/1 -> Q_Latched/1, Unit Delay/1
  D/1 -> Switch/3, OR/1
  OR/1 -> AND/1
  AND/1 -> Switch/2
  Enable/!Rst/1 -> AND/2
  Constant/1 -> Switch/1

== system Lib_Piccolo/Ground Detection Systems/WoW Wrapper/Variant Subsystem/Load Cell WoW Model 18/Subsystem/Landing Configuration/Latching Logic/Latch ==
  D : Inport
  Enable/!Rst : Inport  Port=2
  AND : Logic  IconShape=distinctive  AllPortsSameDT=off  OutDataTypeStr=boolean
  Constant : Constant  OutDataTypeStr=boolean
  OR : Logic  Operator=OR  IconShape=distinctive  AllPortsSameDT=off  OutDataTypeStr=boolean
  Switch : Switch  Criteria=u2 > Threshold  Threshold=0.5
  Unit Delay : UnitDelay  SampleTime=-1
  Q_Latched : Outport
  wires:
  Constant/1 -> Switch/1
  Enable/!Rst/1 -> AND/2
  AND/1 -> Switch/2
  OR/1 -> AND/1
  D/1 -> OR/1, Switch/3
  Switch/1 -> Unit Delay/1, Q_Latched/1
  Unit Delay/1 -> OR/2

== system Lib_Piccolo/Ground Detection Systems/WoW Wrapper/Variant Subsystem/Load Cell WoW Model 18/Subsystem/Landing Configuration/Latching Logic/Primary Latch Timer ==
  Enable/!Rst : Inport
  Compare To Constant1 : simulink/Logic and Bit Operations/Compare To Constant  relop=>  const=0  OutDataTypeStr=uint8
  Compare To Constant2 : simulink/Logic and Bit Operations/Compare To Constant  relop=>=  const=period  OutDataTypeStr=boolean
  Compare To Constant3 : simulink/Logic and Bit Operations/Compare To Constant  relop===  const=0  OutDataTypeStr=boolean
  Discrete-Time Integrator : DiscreteIntegrator  ExternalReset=level  SampleTime=-1  OutDataTypeStr=double  ICPrevOutput=DiscIntNeverNeededParam  ICPrevScaledInput=DiscIntNeverNeededParam
  Expired : Outport
  wires:
  Compare To Constant1/1 -> Discrete-Time Integrator/1
  Compare To Constant2/1 -> Expired/1
  Discrete-Time Integrator/1 -> Compare To Constant2/1
  Enable/!Rst/1 -> Compare To Constant1/1, Compare To Constant3/1
  Compare To Constant3/1 -> Discrete-Time Integrator/2

== system Lib_Piccolo/Ground Detection Systems/WoW Wrapper/Variant Subsystem/Load Cell WoW Model 18/Subsystem/Landing Configuration/Timeout Logic/1-Wheel Timeout ==
  Enable/!Rst : Inport
  Compare To Constant1 : simulink/Logic and Bit Operations/Compare To Constant  relop=>  const=0  OutDataTypeStr=uint8
  Compare To Constant2 : simulink/Logic and Bit Operations/Compare To Constant  relop=>=  const=period  OutDataTypeStr=boolean
  Compare To Constant3 : simulink/Logic and Bit Operations/Compare To Constant  relop===  const=0  OutDataTypeStr=boolean
  Discrete-Time Integrator : DiscreteIntegrator  ExternalReset=level  SampleTime=-1  OutDataTypeStr=double  ICPrevOutput=DiscIntNeverNeededParam  ICPrevScaledInput=DiscIntNeverNeededParam
  Expired : Outport
  wires:
  Compare To Constant1/1 -> Discrete-Time Integrator/1
  Compare To Constant2/1 -> Expired/1
  Discrete-Time Integrator/1 -> Compare To Constant2/1
  Enable/!Rst/1 -> Compare To Constant1/1, Compare To Constant3/1
  Compare To Constant3/1 -> Discrete-Time Integrator/2

== system Lib_Piccolo/Ground Detection Systems/WoW Wrapper/Variant Subsystem/Load Cell WoW Model 20/WOW Module/Landing Configuration/Latching Logic/Latch ==
  D : Inport
  Enable/!Rst : Inport  Port=2
  AND : Logic  IconShape=distinctive  AllPortsSameDT=off  OutDataTypeStr=boolean
  Constant : Constant  OutDataTypeStr=boolean
  OR : Logic  Operator=OR  IconShape=distinctive  AllPortsSameDT=off  OutDataTypeStr=boolean
  Switch : Switch  Criteria=u2 > Threshold  Threshold=0.5
  Unit Delay : UnitDelay  SampleTime=-1
  Q_Latched : Outport
  wires:
  Constant/1 -> Switch/1
  Enable/!Rst/1 -> AND/2
  AND/1 -> Switch/2
  OR/1 -> AND/1
  D/1 -> OR/1, Switch/3
  Switch/1 -> Unit Delay/1, Q_Latched/1
  Unit Delay/1 -> OR/2

== system Lib_Piccolo/Ground Detection Systems/WoW Wrapper/Variant Subsystem/Load Cell WoW Model 20/WOW Module/Landing Configuration/Latching Logic/Primary Latch Timer ==
  Enable/!Rst : Inport
  Compare To Constant1 : simulink/Logic and Bit Operations/Compare To Constant  relop=>  const=0  OutDataTypeStr=uint8
  Compare To Constant2 : simulink/Logic and Bit Operations/Compare To Constant  relop=>=  const=period  OutDataTypeStr=boolean
  Compare To Constant3 : simulink/Logic and Bit Operations/Compare To Constant  relop===  const=0  OutDataTypeStr=boolean
  Discrete-Time Integrator : DiscreteIntegrator  ExternalReset=level  SampleTime=-1  OutDataTypeStr=double  ICPrevOutput=DiscIntNeverNeededParam  ICPrevScaledInput=DiscIntNeverNeededParam
  Expired : Outport
  wires:
  Compare To Constant1/1 -> Discrete-Time Integrator/1
  Compare To Constant2/1 -> Expired/1
  Discrete-Time Integrator/1 -> Compare To Constant2/1
  Enable/!Rst/1 -> Compare To Constant1/1, Compare To Constant3/1
  Compare To Constant3/1 -> Discrete-Time Integrator/2

== system Lib_Piccolo/Ground Detection Systems/WoW Wrapper/Variant Subsystem/Load Cell WoW Model 20/WOW Module/Landing Configuration/Timeout Logic/1-Wheel Timeout ==
  Enable/!Rst : Inport
  Compare To Constant1 : simulink/Logic and Bit Operations/Compare To Constant  relop=>  const=0  OutDataTypeStr=uint8
  Compare To Constant2 : simulink/Logic and Bit Operations/Compare To Constant  relop=>=  const=period  OutDataTypeStr=boolean
  Compare To Constant3 : simulink/Logic and Bit Operations/Compare To Constant  relop===  const=0  OutDataTypeStr=boolean
  Discrete-Time Integrator : DiscreteIntegrator  ExternalReset=level  SampleTime=-1  OutDataTypeStr=double  ICPrevOutput=DiscIntNeverNeededParam  ICPrevScaledInput=DiscIntNeverNeededParam
  Expired : Outport
  wires:
  Compare To Constant1/1 -> Discrete-Time Integrator/1
  Compare To Constant2/1 -> Expired/1
  Discrete-Time Integrator/1 -> Compare To Constant2/1
  Enable/!Rst/1 -> Compare To Constant1/1, Compare To Constant3/1
  Compare To Constant3/1 -> Discrete-Time Integrator/2

== system Lib_Piccolo/Ground Detection Systems/WoW Wrapper/Variant Subsystem/Load Cell WoW Model 20/WOW Module/Subsystem/Comms Timeout Logic/FLAG Timeout Counter ==
  Trigger/!Rst : Inport  OutDataTypeStr=boolean
  x0 : Inport  Port=2
  Compare To Constant : simulink/Logic and Bit Operations/Compare To Constant  relop=>=  const=SensorModel.WOW.Cell.FLAG_TIMEOUT_COUNTS  OutDataTypeStr=boolean
  Custom Counter : Subsystem
  Limit Count : $bdroot/Ground Detection Systems/WoW Wrapper/Variant Subsystem/Load Cell WoW Model 20/WOW Module/Subsystem/Comms Timeout Logic/LOAD Timeout Counter/Limit Count  SystemSampleTime=-1
  NOT : Logic  Operator=NOT  IconShape=distinctive  AllPortsSameDT=off  OutDataTypeStr=boolean
  TIMEOUT : Outport
  wires:
  Custom Counter/1(Cnt) -> Compare To Constant/1  "Cnt"
  Trigger/!Rst/1 -> Limit Count/2, NOT/1
  Compare To Constant/1 -> Limit Count/1, TIMEOUT/1
  x0/1 -> Custom Counter/3(Init)
  Limit Count/1 -> Custom Counter/1(Inc)
  NOT/1 -> Custom Counter/2(Rst)

== system Lib_Piccolo/Ground Detection Systems/WoW Wrapper/Variant Subsystem/Load Cell WoW Model 20/WOW Module/Subsystem/Comms Timeout Logic/LOAD Timeout Counter ==
  Trigger/!Rst : Inport  OutDataTypeStr=boolean
  x0 : Inport  Port=2
  Compare To Constant : simulink/Logic and Bit Operations/Compare To Constant  relop=>=  const=SensorModel.WOW.Cell.LOAD_TIMEOUT_COUNTS  OutDataTypeStr=boolean
  Custom Counter : Subsystem
  Limit Count : Subsystem
  NOT : Logic  Operator=NOT  IconShape=distinctive  AllPortsSameDT=off  OutDataTypeStr=boolean
  TIMEOUT : Outport
  wires:
  NOT/1 -> Custom Counter/2(Rst)
  Limit Count/1(Inc) -> Custom Counter/1(Inc)
  x0/1 -> Custom Counter/3(Init)
  Compare To Constant/1 -> Limit Count/1(Timeout), TIMEOUT/1
  Custom Counter/1(Cnt) -> Compare To Constant/1  "Cnt"
  Trigger/!Rst/1 -> Limit Count/2(Trigger), NOT/1

== system Lib_Piccolo/Ground Detection Systems/WoW Wrapper/Variant Subsystem/Load Cell WoW Model 20/WOW Module/Subsystem/Comms Timeout Logic/Latch ==
  D : Inport
  Enable/!Rst : Inport  Port=2
  AND : Logic  IconShape=distinctive  AllPortsSameDT=off  OutDataTypeStr=boolean
  Constant : Constant  OutDataTypeStr=boolean
  OR : Logic  Operator=OR  IconShape=distinctive  AllPortsSameDT=off  OutDataTypeStr=boolean
  Switch : Switch  Criteria=u2 > Threshold  Threshold=0.5
  Unit Delay : UnitDelay  SampleTime=-1
  Q_Latched : Outport
  wires:
  Constant/1 -> Switch/1
  Enable/!Rst/1 -> AND/2
  AND/1 -> Switch/2
  OR/1 -> AND/1
  D/1 -> OR/1, Switch/3
  Switch/1 -> Unit Delay/1, Q_Latched/1
  Unit Delay/1 -> OR/2

== system Lib_Piccolo/Ground Detection Systems/WoW Wrapper/Variant Subsystem/Load Cell WoW Model 20/WOW Module/Subsystem/Comms Timeout Logic/Reset Value Selector ==
  Init : Inport  OutDataTypeStr=boolean
  Constant : Constant  Value=SensorModel.WOW.Cell.LOAD_TIMEOUT_COUNTS  OutDataTypeStr=uint8
  Constant1 : Constant  Value=SensorModel.WOW.Cell.FLAG_TIMEOUT_COUNTS  OutDataTypeStr=uint8
  Constant2 : Constant  Value=0  OutDataTypeStr=uint8
  Constant3 : Constant  Value=0  OutDataTypeStr=uint8
  Switch : Switch  Criteria=u2 > Threshold  Threshold=0.5
  Switch1 : Switch  Criteria=u2 > Threshold  Threshold=0.5
  Reset Value LOAD : Outport  OutDataTypeStr=uint8
  Reset Value FLAG : Outport  Port=2  OutDataTypeStr=uint8
  wires:
  Init/1 -> Switch1/2, Switch/2
  Constant/1 -> Switch/1
  Constant1/1 -> Switch1/1
  Switch/1 -> Reset Value LOAD/1
  Switch1/1 -> Reset Value FLAG/1
  Constant2/1 -> Switch1/3
  Constant3/1 -> Switch/3

== system Lib_Piccolo/Ground Detection Systems/WoW Wrapper/Variant Subsystem/Load Cell WoW Model 20/WOW Module/Subsystem/Health Check/DSC FLAG Decode ==
  MGR FLAG Word : Inport  OutDataTypeStr=uint16
  MGL FLAG Word : Inport  Port=2  OutDataTypeStr=uint16
  NG FLAG Word : Inport  Port=3  OutDataTypeStr=uint16
  Bus Creator : BusCreator  Inputs=TEMPUR,TEMPOR,ECOMUR,ECOMOR,CRAWUR,CRAWOR,SYSUR,SYSOR,LCINTEG,WDRST,BRWNOUT,REBOOT,LOWER_FLAGS  OutDataTypeStr=Bus: FLAG_SIGNAL_BUS  NonVirtualBus=on
  Bus Creator1 : BusCreator  Inputs=TEMPUR,TEMPOR,ECOMUR,ECOMOR,CRAWUR,CRAWOR,SYSUR,SYSOR,LCINTEG,WDRST,BRWNOUT,REBOOT,LOWER_FLAGS  OutDataTypeStr=Bus: FLAG_SIGNAL_BUS  NonVirtualBus=on
  Bus Creator2 : BusCreator  Inputs=TEMPUR,TEMPOR,ECOMUR,ECOMOR,CRAWUR,CRAWOR,SYSUR,SYSOR,LCINTEG,WDRST,BRWNOUT,REBOOT,LOWER_FLAGS  OutDataTypeStr=Bus: FLAG_SIGNAL_BUS  NonVirtualBus=on
  Extract Flags MGL : $bdroot/Ground Detection Systems/WoW Wrapper/Variant Subsystem/Load Cell WoW Model 20/WOW Module/Subsystem/Health Check/DSC FLAG Decode/Extract Flags MGR  SystemSampleTime=-1
  Extract Flags MGR : Subsystem
  Extract Flags NG : $bdroot/Ground Detection Systems/WoW Wrapper/Variant Subsystem/Load Cell WoW Model 20/WOW Module/Subsystem/Health Check/DSC FLAG Decode/Extract Flags MGR  SystemSampleTime=-1
  OR : Logic  Operator=OR  Inputs=3  IconShape=distinctive  AllPortsSameDT=off  OutDataTypeStr=boolean
  OR1 : Logic  Operator=OR  Inputs=3  IconShape=distinctive  AllPortsSameDT=off  OutDataTypeStr=boolean
  OR2 : Logic  Operator=OR  Inputs=3  IconShape=distinctive  AllPortsSameDT=off  OutDataTypeStr=boolean
  Persistence Counter : Subsystem
  Persistence Counter1 : $bdroot/Ground Detection Systems/WoW Wrapper/Variant Subsystem/Load Cell WoW Model 20/WOW Module/Subsystem/Health Check/DSC FLAG Decode/Persistence Counter  SystemSampleTime=-1
  Persistence Counter2 : $bdroot/Ground Detection Systems/WoW Wrapper/Variant Subsystem/Load Cell WoW Model 20/WOW Module/Subsystem/Health Check/DSC FLAG Decode/Persistence Counter  SystemSampleTime=-1
  MGR_FLAG_RESET : Outport
  MGL_FLAG_RESET : Outport  Port=2
  NG_FLAG_RESET : Outport  Port=3
  MGR_FLAGS : Outport  Port=4
  MGL_FLAGS : Outport  Port=5
  NG_FLAGS : Outport  Port=6
  wires:
  MGL FLAG Word/1 -> Extract Flags MGL/1
  NG FLAG Word/1 -> Extract Flags NG/1
  Extract Flags MGR/4(ECOMOR) -> Bus Creator/4, OR/2  "ECOMOR"
  Extract Flags MGR/13(LOWER_FLAGS) -> Bus Creator/13  "LOWER_FLAGS"
  Bus Creator/1 -> MGR_FLAGS/1
  Extract Flags MGR/11(BRWNOUT) -> Bus Creator/11  "BRWNOUT"
  Extract Flags MGR/10(WDRST) -> Bus Creator/10  "WDRST"
  Extract Flags MGR/8(SYSOR) -> Bus Creator/8  "SYSOR"
  Extract Flags MGR/12(REBOOT) -> Bus Creator/12  "REBOOT"
  Extract Flags MGR/1(TEMPUR) -> Bus Creator/1  "TEMPUR"
  Extract Flags MGR/9(LCINTEG) -> Bus Creator/9, OR/3  "LCINTEG"
  OR/1 -> Persistence Counter/1(Trigger/!Rst)
  Extract Flags MGR/2(TEMPOR) -> Bus Creator/2  "TEMPOR"
  Extract Flags MGR/6(CRAWOR) -> Bus Creator/6  "CRAWOR"
  Extract Flags MGR/5(CRAWUR) -> Bus Creator/5  "CRAWUR"
  Extract Flags MGR/7(SYSUR) -> Bus Creator/7  "SYSUR"
  Extract Flags MGR/3(ECOMUR) -> Bus Creator/3, OR/1  "ECOMUR"
  MGR FLAG Word/1 -> Extract Flags MGR/1(Flag Word)
  Extract Flags MGL/1 -> Bus Creator1/1  "TEMPUR"
  Extract Flags MGL/12 -> Bus Creator1/12  "REBOOT"
  Extract Flags MGL/8 -> Bus Creator1/8  "SYSOR"
  Extract Flags MGL/10 -> Bus Creator1/10  "WDRST"
  Extract Flags MGL/5 -> Bus Creator1/5  "CRAWUR"
  Extract Flags MGL/2 -> Bus Creator1/2  "TEMPOR"
  OR1/1 -> Persistence Counter1/1
  Extract Flags MGL/9 -> Bus Creator1/9, OR1/3  "LCINTEG"
  Bus Creator1/1 -> MGL_FLAGS/1
  Extract Flags MGL/6 -> Bus Creator1/6  "CRAWOR"
  Extract Flags MGL/7 -> Bus Creator1/7  "SYSUR"
  Extract Flags MGL/13 -> Bus Creator1/13  "LOWER_FLAGS"
  Extract Flags MGL/11 -> Bus Creator1/11  "BRWNOUT"
  Extract Flags MGL/4 -> Bus Creator1/4, OR1/2  "ECOMOR"
  Extract Flags MGL/3 -> Bus Creator1/3, OR1/1  "ECOMUR"
  Extract Flags NG/1 -> Bus Creator2/1  "TEMPUR"
  Extract Flags NG/12 -> Bus Creator2/12  "REBOOT"
  Extract Flags NG/8 -> Bus Creator2/8  "SYSOR"
  Extract Flags NG/10 -> Bus Creator2/10  "WDRST"
  Extract Flags NG/5 -> Bus Creator2/5  "CRAWUR"
  Extract Flags NG/2 -> Bus Creator2/2  "TEMPOR"
  OR2/1 -> Persistence Counter2/1
  Extract Flags NG/9 -> Bus Creator2/9, OR2/3  "LCINTEG"
  Bus Creator2/1 -> NG_FLAGS/1
  Extract Flags NG/6 -> Bus Creator2/6  "CRAWOR"
  Extract Flags NG/7 -> Bus Creator2/7  "SYSUR"
  Extract Flags NG/13 -> Bus Creator2/13  "LOWER_FLAGS"
  Extract Flags NG/11 -> Bus Creator2/11  "BRWNOUT"
  Extract Flags NG/4 -> Bus Creator2/4, OR2/2  "ECOMOR"
  Extract Flags NG/3 -> Bus Creator2/3, OR2/1  "ECOMUR"
  Persistence Counter/1(TIMEOUT) -> MGR_FLAG_RESET/1
  Persistence Counter1/1 -> MGL_FLAG_RESET/1
  Persistence Counter2/1 -> NG_FLAG_RESET/1
